simulink model "current_limiting_B_test"  (R2018b)
settings: Solver=VariableStepAuto  StartTime=0.0  StopTime=5  RelTol=1e-3
PreLoadFcn:
  | load_system('../simulink_reference_models/test_sequence_lib');
InitFcn:
  | close all
  | clear all
  | 
  | T_CNTL = 1/5e3;
  | 
  | VLL_NOM = 35e3;
  | F_NOM = 60;
undefined symbols (not defined in the file): j
libraries: simulink x14
settings Model: SimulationMode=rapid-accelerator  Creator=HussamAlatrash  LastModifiedBy=ahhei
settings DataIOCC: ReturnWorkspaceOutputs=on
settings DebuggingCC: UnconnectedInputMsg=none  UnconnectedOutputMsg=none  UnconnectedLineMsg=none
settings ModelReferenceCC: EnableRefExpFcnMdlSchedulingChecks=off
settings RTWCC: Description=Generic Real-Time Target
settings ConfigComp: CovBoundaryAbsTol=1.0e-5

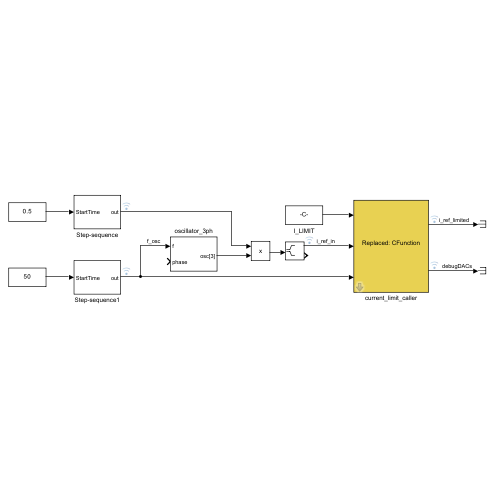
[thumbnail: Simulink's stored preview of the top-level diagram]
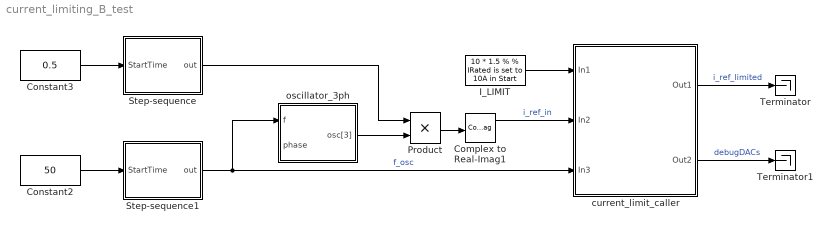
== system current_limiting_B_test ==
  Complex to Real-Imag1 : ComplexToRealImag
  Constant2 : Constant  Value=50
  Constant3 : Constant  Value=0.5
  I_LIMIT : Constant  Value=10 * 1.5 % % IRated is set to 10A in Start
  Product : Product
  Step-sequence : Subsystem
  Step-sequence1 : Subsystem
  Terminator : Terminator
  Terminator1 : Terminator
  current_limit_caller : Subsystem  Description=Replaced Block  mask(Replaced Block){}
      mask help: This block has been replaced with an empty subsystem because it used functionality that is unavailable in Simulink R2018b.
      mask Display: fprintf('Replaced: %s\n','CFunction')
  oscillator_3ph : Subsystem
  wires:
  current_limit_caller/2(Out2) -> Terminator1/1  "debugDACs"
  current_limit_caller/1(Out1) -> Terminator/1  "i_ref_limited"
  Step-sequence1/1(out) -> oscillator_3ph/1(f), current_limit_caller/3(In3)  "f_osc"
  Constant2/1 -> Step-sequence1/1(StartTime)
  Constant3/1 -> Step-sequence/1(StartTime)
  oscillator_3ph/1(osc[3]) -> Product/2
  Step-sequence/1(out) -> Product/1
  Product/1 -> Complex to Real-Imag1/1
  Complex to Real-Imag1/1 -> current_limit_caller/2(In2)  "i_ref_in"
  I_LIMIT/1 -> current_limit_caller/1(In1)

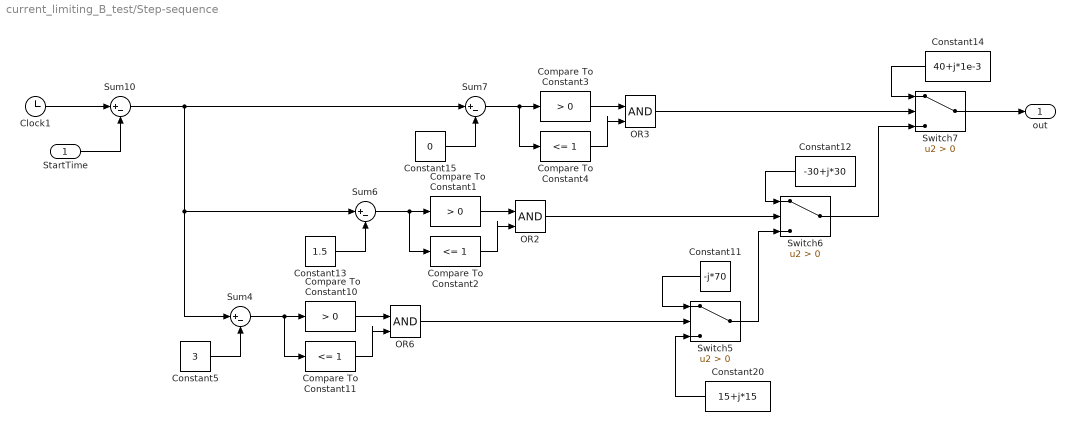
== system current_limiting_B_test/Step-sequence ==
  StartTime : Inport
  Clock1 : Clock
  Compare To Constant1 : simulink/Logic and Bit Operations/Compare To Constant  relop=>  const=0  OutDataTypeStr=boolean
  Compare To Constant10 : simulink/Logic and Bit Operations/Compare To Constant  relop=>  const=0  OutDataTypeStr=boolean
  Compare To Constant11 : simulink/Logic and Bit Operations/Compare To Constant  relop=<=  const=1  OutDataTypeStr=boolean
  Compare To Constant2 : simulink/Logic and Bit Operations/Compare To Constant  relop=<=  const=1  OutDataTypeStr=boolean
  Compare To Constant3 : simulink/Logic and Bit Operations/Compare To Constant  relop=>  const=0  OutDataTypeStr=boolean
  Compare To Constant4 : simulink/Logic and Bit Operations/Compare To Constant  relop=<=  const=1  OutDataTypeStr=boolean
  Constant11 : Constant  Value=-j*70
  Constant12 : Constant  Value=-30+j*30
  Constant13 : Constant  Value=1.5
  Constant14 : Constant  Value=40+j*1e-3
  Constant15 : Constant  Value=0
  Constant20 : Constant  Value=15+j*15
  Constant5 : Constant  Value=3
  OR2 : Logic  IconShape=distinctive  AllPortsSameDT=off  OutDataTypeStr=boolean
  OR3 : Logic  IconShape=distinctive  AllPortsSameDT=off  OutDataTypeStr=boolean
  OR6 : Logic  IconShape=distinctive  AllPortsSameDT=off  OutDataTypeStr=boolean
  Sum{4,6..7,10} (4 alike) : Sum  Inputs=|+-
  Switch5 : Switch  Criteria=u2 > Threshold
  Switch6 : Switch  Criteria=u2 > Threshold
  Switch7 : Switch  Criteria=u2 > Threshold
  out : Outport
  wires:
  Sum4/1 -> Compare To Constant10/1, Compare To Constant11/1
  Constant5/1 -> Sum4/2
  OR6/1 -> Switch5/2
  Compare To Constant10/1 -> OR6/1
  Compare To Constant11/1 -> OR6/2
  Constant11/1 -> Switch5/1
  Switch5/1 -> Switch6/3
  Constant12/1 -> Switch6/1
  Compare To Constant2/1 -> OR2/2
  Compare To Constant1/1 -> OR2/1
  OR2/1 -> Switch6/2
  Constant13/1 -> Sum6/2
  Sum6/1 -> Compare To Constant2/1, Compare To Constant1/1
  Sum7/1 -> Compare To Constant3/1, Compare To Constant4/1
  Constant15/1 -> Sum7/2
  OR3/1 -> Switch7/2
  Compare To Constant3/1 -> OR3/1
  Compare To Constant4/1 -> OR3/2
  Constant14/1 -> Switch7/1
  Switch7/1 -> out/1
  Sum10/1 -> Sum7/1, Sum6/1, Sum4/1
  Clock1/1 -> Sum10/1
  StartTime/1 -> Sum10/2
  Switch6/1 -> Switch7/3
  Constant20/1 -> Switch5/3

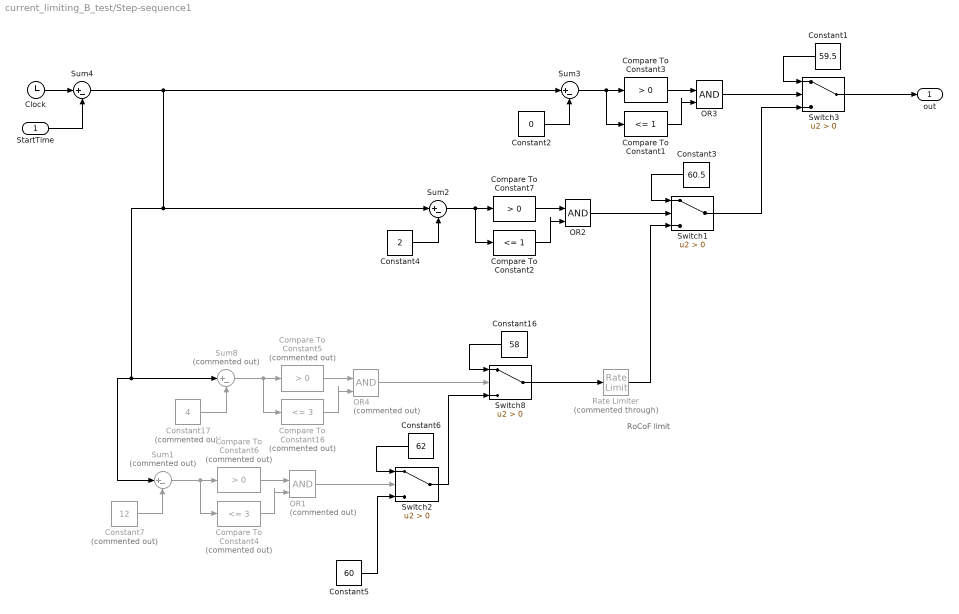
== system current_limiting_B_test/Step-sequence1 ==
  note: RoCoF limit
  StartTime : Inport
  Clock : Clock
  Compare To Constant1 : simulink/Logic and Bit Operations/Compare To Constant  relop=<=  const=1  OutDataTypeStr=boolean
  Compare To Constant16 : simulink/Logic and Bit Operations/Compare To Constant  Commented=on  relop=<=  const=3  OutDataTypeStr=boolean
  Compare To Constant2 : simulink/Logic and Bit Operations/Compare To Constant  relop=<=  const=1  OutDataTypeStr=boolean
  Compare To Constant3 : simulink/Logic and Bit Operations/Compare To Constant  relop=>  const=0  OutDataTypeStr=boolean
  Compare To Constant4 : simulink/Logic and Bit Operations/Compare To Constant  Commented=on  relop=<=  const=3  OutDataTypeStr=boolean
  Compare To Constant5 : simulink/Logic and Bit Operations/Compare To Constant  Commented=on  relop=>  const=0  OutDataTypeStr=boolean
  Compare To Constant6 : simulink/Logic and Bit Operations/Compare To Constant  Commented=on  relop=>  const=0  OutDataTypeStr=boolean
  Compare To Constant7 : simulink/Logic and Bit Operations/Compare To Constant  relop=>  const=0  OutDataTypeStr=boolean
  Constant1 : Constant  Value=59.5
  Constant16 : Constant  Value=58
  Constant17 : Constant  Commented=on  Value=4
  Constant2 : Constant  Value=0
  Constant3 : Constant  Value=60.5
  Constant4 : Constant  Value=2
  Constant5 : Constant  Value=60
  Constant6 : Constant  Value=62
  Constant7 : Constant  Commented=on  Value=12
  OR1 : Logic  Commented=on  IconShape=distinctive  AllPortsSameDT=off  OutDataTypeStr=boolean
  OR2 : Logic  IconShape=distinctive  AllPortsSameDT=off  OutDataTypeStr=boolean
  OR3 : Logic  IconShape=distinctive  AllPortsSameDT=off  OutDataTypeStr=boolean
  OR4 : Logic  Commented=on  IconShape=distinctive  AllPortsSameDT=off  OutDataTypeStr=boolean
  Rate Limiter : RateLimiter  Commented=through  RisingSlewLimit=5  FallingSlewLimit=-5  SampleTimeMode=inherited  InitialCondition=60
  Sum1 : Sum  Commented=on  Inputs=|+-
  Sum2 : Sum  Inputs=|+-
  Sum3 : Sum  Inputs=|+-
  Sum4 : Sum  Inputs=|+-
  Sum8 : Sum  Commented=on  Inputs=|+-
  Switch{1..3,8} (4 alike) : Switch  Criteria=u2 > Threshold
  out : Outport
  wires:
  Switch2/1 -> Switch8/3
  Constant16/1 -> Switch8/1
  OR4/1 -> Switch8/2
  Compare To Constant5/1 -> OR4/1
  Sum8/1 -> Compare To Constant5/1, Compare To Constant16/1
  Constant17/1 -> Sum8/2
  Compare To Constant16/1 -> OR4/2
  Switch8/1 -> Rate Limiter/1
  Constant5/1 -> Switch2/3
  Constant6/1 -> Switch2/1
  OR1/1 -> Switch2/2
  Compare To Constant6/1 -> OR1/1
  Sum1/1 -> Compare To Constant6/1, Compare To Constant4/1
  Constant7/1 -> Sum1/2
  Compare To Constant4/1 -> OR1/2
  Compare To Constant2/1 -> OR2/2
  Constant4/1 -> Sum2/2
  Sum2/1 -> Compare To Constant2/1, Compare To Constant7/1
  Compare To Constant7/1 -> OR2/1
  OR2/1 -> Switch1/2
  Constant3/1 -> Switch1/1
  Rate Limiter/1 -> Switch1/3
  Switch3/1 -> out/1
  Compare To Constant1/1 -> OR3/2
  Constant2/1 -> Sum3/2
  Sum3/1 -> Compare To Constant1/1, Compare To Constant3/1
  Compare To Constant3/1 -> OR3/1
  OR3/1 -> Switch3/2
  Constant1/1 -> Switch3/1
  Sum4/1 -> Sum1/1, Sum8/1, Sum2/1, Sum3/1
  Switch1/1 -> Switch3/3
  Clock/1 -> Sum4/1
  StartTime/1 -> Sum4/2

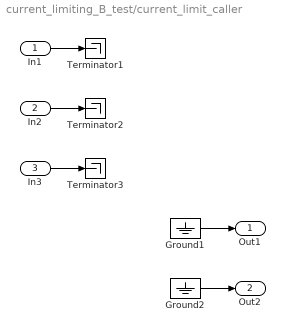
== system current_limiting_B_test/current_limit_caller ==
  In1 : Inport
  In2 : Inport  Port=2
  In3 : Inport  Port=3
  Ground1 : Ground
  Ground2 : Ground
  Terminator1 : Terminator
  Terminator2 : Terminator
  Terminator3 : Terminator
  Out1 : Outport
  Out2 : Outport  Port=2
  wires:
  Ground2/1 -> Out2/1
  Ground1/1 -> Out1/1
  In3/1 -> Terminator3/1
  In2/1 -> Terminator2/1
  In1/1 -> Terminator1/1

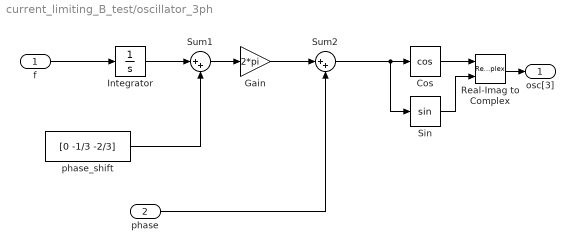
== system current_limiting_B_test/oscillator_3ph ==
  f : Inport
  phase : Inport  Port=2
  Cos : Trigonometry  Operator=cos
  Gain : Gain  Gain=2*pi
  Integrator : Integrator  InitialCondition=0.25
  Real-Imag to Complex : RealImagToComplex
  Sin : Trigonometry
  Sum1 : Sum  Inputs=|++
  Sum2 : Sum  Inputs=|++
  phase_shift : Constant  Value=[0 -1/3 -2/3]
  osc[3] : Outport
  wires:
  Sum1/1 -> Gain/1
  Sin/1 -> Real-Imag to Complex/2
  Integrator/1 -> Sum1/1
  Sum2/1 -> Sin/1, Cos/1
  Cos/1 -> Real-Imag to Complex/1
  Real-Imag to Complex/1 -> osc[3]/1
  f/1 -> Integrator/1
  phase_shift/1 -> Sum1/2
  phase/1 -> Sum2/2
  Gain/1 -> Sum2/1
